simulink model "turbo_controller"  (R2025a)
settings: Solver=FixedStepAuto  StartTime=0.0  StopTime=inf  FixedStep=0.001  RelTol=1e-3
PostLoadFcn:
  | % 自动定位同目录CubeMX文件；不需要外部初始化脚本。
  | codertarget.data.setParameterValue('turbo_controller','STM32CubeMX.ProjectFile',fullfile(fileparts(get_param('turbo_controller','FileName')),'turbo_f407.ioc'));
InitFcn:
  | % 中文说明：按原控制器字段与类型创建三组接口总线；控制参数已内嵌。
  | tc_names=["EValve_Cycle" "EValve_Open" "Eblast_Cycle" "Eblast_Open" "Motor_Cycle" "Motor_Open" "EValve_Enable" "Eblast_Enable" "Motor_Enable" "SWO_Firework" "SWO_BleedAir" "EngineState" "Flag_ECUReset_Clear" "Flag_ECUReset_Save" "Flag_Reset_Enable" "Accelerator" "Nc_dem" "Nc"]; tc_types=["uint16" "uint16" "uint16" "uint16" "uint16" "uint16" "uint8" "uint8" "uint8" "uint8" "uint8" "uint8" "uint8" "uint8" "uint8" "single" "single" "single"];
  | for tc_k=1:numel(tc_names)
  |  tc_e(tc_k)=Simulink.BusElement; tc_e(tc_k).Name=char(tc_names(tc_k)); tc_e(tc_k).DataType=char(tc_types(tc_k));
  | end
  | EngineControl_Out=Simulink.Bus; EngineControl_Out.DataScope='Exported'; EngineControl_Out.Elements=tc_e;
  | clear tc_e tc_names tc_types tc_k
  | tc_names=["savedata1" "savedata2" "savedata3" "savedata4" "savedata5" "savedata6" "savedata7" "savedata8" "savedata9" "savedata10" "savedata11" "savedata12" "savedata13" "savedata14" "savedata15" "savedata16" "savedata17" "savedata18" "savedata19" "savedata20" "savedata21" "savedata22" "savedata23" "savedata24" "savedata25"]; tc_types=["single" "single" "single" "single" "single" "single" "single" "single" "single" "single" "single" "single" "single" "single" "single" "single" "single" "single" "single" "single" "single" "single" "single" "single" "single"];
  | for tc_k=1:numel(tc_names)
  |  tc_e(tc_k)=Simulink.BusElement; tc_e(tc_k).Name=char(tc_names(tc_k)); tc_e(tc_k).DataType=char(tc_types(tc_k));
  | end
  | SaveData_Out=Simulink.Bus; SaveData_Out.DataScope='Exported'; SaveData_Out.Elements=tc_e;
  | clear tc_e tc_names tc_types tc_k
  | tc_names=["senddata1" "senddata2" "senddata3" "senddata4" "senddata5" "senddata6" "senddata7" "senddata8" "senddata9" "senddata10" "senddata11" "senddata12" "senddata13" "senddata14" "senddata15" "senddata16" "senddata17" "senddata18" "senddata19" "senddata20" "senddata21" "senddata22" "senddata23" "senddata24" "senddata25" "senddata26" "senddata27" "senddata28" "senddata29"]; tc_types=["uint8" "uint8" "uint8" "uint8" "uint8" "uint8" "uint8" "uint8" "uint8" "uint8" "uint8" "uint8" "uint8" "uint8" "uint8" "uint8" "uint8" "uint8" "uint8" "uint8" "uint8" "uint8" "uint8" "uint8" "uint8" "uint8" "uint8" "uint8" "uint8"];
  | for tc_k=1:numel(tc_names)
  |  tc_e(tc_k)=Simulink.BusElement; tc_e(tc_k).Name=char(tc_names(tc_k)); tc_e(tc_k).DataType=char(tc_types(tc_k));
  | end
  | SendData_Out=Simulink.Bus; SendData_Out.DataScope='Exported'; SendData_Out.Elements=tc_e;
  | clear tc_e tc_names tc_types tc_k
  | 
  | % 以下为接口中文说明；只设置描述，不改变数值或数据类型。
  | EngineControl_Out.Description='执行控制输出（阀、电机、点火、状态及复位请求）';
  | tc_cn=["EValve_Cycle（主油阀周期计数（每计数2毫秒））" "EValve_Open（主油阀开通计数（每计数2毫秒））" "Eblast_Cycle（副油阀周期计数（每计数2毫秒））" "Eblast_Open（副油阀开通计数（每计数2毫秒））" "Motor_Cycle（起动电机周期计数）" "Motor_Open（起动电机开通计数）" "EValve_Enable（主油阀驱动使能）" "Eblast_Enable（副油阀驱动使能）" "Motor_Enable（起动电机使能）" "SWO_Firework（点火器使能（1开））" "SWO_BleedAir（引气阀使能（1开））" "EngineState（发动机状态）" "Flag_ECUReset_Clear（清除复位恢复状态请求）" "Flag_ECUReset_Save（保存复位恢复数据请求）" "Flag_Reset_Enable（处理器软件复位请求）" "Accelerator（油门／油泵给定控制量）" "Nc_dem（控制目标转速）" "Nc（发动机反馈转速（转每分））"];
  | tc_elements=EngineControl_Out.Elements;
  | for tc_k=1:numel(tc_cn)
  |  tc_elements(tc_k).Description=char(tc_cn(tc_k));
  | end
  | EngineControl_Out.Elements=tc_elements;
  | clear tc_cn tc_elements tc_k
  | SaveData_Out.Description='25项运行记录；字段含义按当前模型数据来源解释';
  | tc_cn=["savedata1（指令回显记录）" "savedata2（入口总温记录（℃））" "savedata3（电源电压记录）" "savedata4（排气温度记录（℃））" "savedata5（标定燃油压力记录）" "savedata6（副油阀占空比记录（％））" "savedata7（主油阀占空比记录（％））" "savedata8（温度修正转速记录）" "savedata9（开关输出及反馈位域）" "savedata10（物理转速记录）" "savedata11（油泵目标给定原始值）" "savedata12（起动电机占空比记录（％））" "savedata13（发动机状态码记录）" "savedata14（故障告警位域记录）" "savedata15（模型记录帧序号）" "savedata16（处理器温度记录（℃））" "savedata17（装订转速记录（沿用旧电源字段名））" "savedata18（导航高度记录）" "savedata19（飞行空速记录）" "savedata20（主阀旧记录位（恒零保留））" "savedata21（第21项保留记录（恒零））" "savedata22（保留记录项22）" "savedata23（保留记录项23）" "savedata24（保留记录项24）" "savedata25（保留记录项25）"];
  | tc_elements=SaveData_Out.Elements;
  | for tc_k=1:numel(tc_cn)
  |  tc_elements(tc_k).Description=char(tc_cn(tc_k));
  | end
  | SaveData_Out.Elements=tc_elements;
  | clear tc_cn tc_elements tc_k
  | SendData_Out.Description='29字段回传及外设命令接口；板端上位机帧只取第3至27字段';
  | tc_cn=["senddata1（回传发送允许标志（不直接上线路））" "senddata2（回传载荷长度25字节）" "senddata3（回传指令回显字节）" "senddata4（总温编码字节（℃＋80））" "senddata5（电源电压编码字节）" "senddata6（排温编码高字节）" "senddata7（排温编码低字节）" "senddata8（燃油压力编码高字节）" "senddata9（燃油压力编码低字节）" "senddata10（副油阀占空比字节（％））" "senddata11（主油阀占空比字节（％））" "senddata12（修正转速编码高字节）" "senddata13（修正转速编码低字节）" "senddata14（驱动及反馈状态位域）" "senddata15（物理转速编码高字节）" "senddata16（物理转速编码低字节）" "senddata17（油泵目标给定高字节（串口二使用））" "senddata18（油泵目标给定低字节（串口二使用））" "senddata19（起动电机占空比命令（串口一使用））" "senddata20（发动机状态码字节）" "senddata21（故障告警位域字节）" "senddata22（帧序号占位（板端另行填写））" "senddata23（处理器温度编码（℃＋50））" "senddata24（控制目标转速编码高字节）" "senddata25（控制目标转速编码低字节）" "senddata26（占位字节（板端改填实测泵速高字节））" "senddata27（占位字节（板端改填实测泵速低字节））" "senddata28（装订转速高字节（本板未发送））" "senddata29（装订转速低字节（本板未发送））"];
  | tc_elements=SendData_Out.Elements;
  | for tc_k=1:numel(tc_cn)
  |  tc_elements(tc_k).Description=char(tc_cn(tc_k));
  | end
  | SendData_Out.Elements=tc_elements;
  | clear tc_cn tc_elements tc_k
  | 
  | 
  | % FRAM模块化事务：接口类型和上电初始状态，随模型保存，无外部初始化文件。
  | clear FM_elements
  | FM_elements(1)=Simulink.BusElement;FM_elements(1).Name='phase';FM_elements(1).DataType='uint8';FM_elements(1).Dimensions=[1 1];FM_elements(1).Description='phase（当前事务阶段）';
  | FM_elements(2)=Simulink.BusElement;FM_elements(2).Name='a';FM_elements(2).DataType='uint8';FM_elements(2).Dimensions=[64 1];FM_elements(2).Description='a（启动时缓存的首区64字节）';
  | FM_elements(3)=Simulink.BusElement;FM_elements(3).Name='active';FM_elements(3).DataType='uint16';FM_elements(3).Dimensions=[1 1];FM_elements(3).Description='active（当前有效记录区地址）';
  | FM_elements(4)=Simulink.BusElement;FM_elements(4).Name='generation';FM_elements(4).DataType='uint32';FM_elements(4).Dimensions=[1 1];FM_elements(4).Description='generation（当前有效记录代号）';
  | FM_elements(5)=Simulink.BusElement;FM_elements(5).Name='record';FM_elements(5).DataType='uint8';FM_elements(5).Dimensions=[64 1];FM_elements(5).Description='record（本次冻结的待写记录）';
  | FM_elements(6)=Simulink.BusElement;FM_elements(6).Name='addr';FM_elements(6).DataType='uint16';FM_elements(6).Dimensions=[1 1];FM_elements(6).Description='addr（本次备用写入地址）';
  | FM_elements(7)=Simulink.BusElement;FM_elements(7).Name='lastSave';FM_elements(7).DataType='single';FM_elements(7).Dimensions=[1 1];FM_elements(7).Description='lastSave（上次开始保存的秒数）';
  | FM_elements(8)=Simulink.BusElement;FM_elements(8).Name='lastState';FM_elements(8).DataType='uint8';FM_elements(8).Dimensions=[1 1];FM_elements(8).Description='lastState（上次保存时的发动机状态）';
  | FM_elements(9)=Simulink.BusElement;FM_elements(9).Name='boot';FM_elements(9).DataType='boolean';FM_elements(9).Dimensions=[1 1];FM_elements(9).Description='boot（启动记录是否允许恢复）';
  | FM_elements(10)=Simulink.BusElement;FM_elements(10).Name='consumed';FM_elements(10).DataType='boolean';FM_elements(10).Dimensions=[1 1];FM_elements(10).Description='consumed（本次启动恢复通知是否已发送）';
  | FM_elements(11)=Simulink.BusElement;FM_elements(11).Name='payload';FM_elements(11).DataType='uint8';FM_elements(11).Dimensions=[20 1];FM_elements(11).Description='payload（当前20字节恢复内容）';
  | ... (+35 lines)
model workspace (MAT data in the model file):
  CRC16_Table_Reference = [0 4129 8258 12387 16516 20645 24774 28903 33032 37161 41290 45419 ... (256 elements, 256x1)]
  PE_Kaer = [0.15402 0.15402 0.12264 0.10076 0.09481 0.07601 0.07111 0.0569 0.05198 0.04926 0.05308 0.04325 ... (13 elements, 1x13)]
  PE_Nr = [21.2982 61.4260372 67.7475458 72.7394382 76.845934 80.6988798 83.8449282 86.6491912 88.9382406 89.178606 91.1938214 93.4068058 ... (13 elements, 1x13)]
  PE_Pump_Translate = 33.5999984741
  PE_RotaSpeed_Translate = 860
  PE_Taer = [0.4939154 0.4939154 0.40780982 0.34066978 0.31622756 0.30405716 0.34300244 0.26785022 0.37393554 0.23914836 0.44563948 0.31044662 ... (13 elements, 1x13)]
  PF_ACCFULLRANGE = 3360
  PF_Flag_ECUReset = 0
  PF_Flag_rx_suc = 1
  PF_Gear_Info = [40000; 45000; 50000; 55000; 57000; 59000; 60000; 61000; 61000; 61000; 61000; 61000]
  PF_K_TiaoJie = 1
  PF_Kpu = 10
  PF_MySet_Rxdata = [0 0 0 0 0 0 0 0 0 0 0 0 ... (50 elements, 50x1)]
  PF_MyUsart1_Rxdata = [0 0 0 0 0 0 0 0 0 0 0 0 ... (50 elements, 50x1)]
  PF_MyUsart2_Rxdata = [0 0 0 0 0 0 0 0 0 0 0 0 ... (50 elements, 50x1)]
  PF_Reset_Information = [0 0 0 0 0 0 0 0 0 0 0 0 ... (20 elements, 20x1)]
  PF_Sensor_X1_T4 = [0 4095]
  PF_Sensor_X2_T4 = [0 1.66666698456]
  PF_Sensor_X3_T4 = [0 504 999 1497 2010 2529 3051 3568 4076 4571 4959]
  PF_Sensor_X_P2 = [0.5 3]
  PF_Sensor_X_Poil = [0.5 3]
  PF_Sensor_X_T1t = [-50 300]
  PF_Sensor_X_Vpower = [0 3]
  PF_Sensor_X_Vpump = [0 3]
  PF_Sensor_Y1_T4 = [0 3]
  PF_Sensor_Y2_T4 = [0 5000]
  PF_Sensor_Y3_T4 = [0 100 200 300 400 500 600 700 800 900 980]
  PF_Sensor_Y_P2 = [0 1000]
  PF_Sensor_Y_Poil = [0 1000]
  PF_Sensor_Y_T1t = [-50 300]
  PF_Sensor_Y_Vpower = [0 33]
  PF_Sensor_Y_Vpump = [0 33]
  PG_CtrlMode_CloseLoop : mpt.Parameter (value not decoded)
  PG_CtrlMode_ManualAcc : mpt.Parameter (value not decoded)
  PG_CtrlMode_Origin : mpt.Parameter (value not decoded)
  PG_CtrlMode_Start : mpt.Parameter (value not decoded)
  PG_CtrlMode_Stop : mpt.Parameter (value not decoded)
  PG_ES_Clp : mpt.Parameter (value not decoded)
  PG_ES_EngStart : mpt.Parameter (value not decoded)
  PG_ES_Manual : mpt.Parameter (value not decoded)
  PG_ES_Origin : mpt.Parameter (value not decoded)
  PG_ES_Stop : mpt.Parameter (value not decoded)
  PG_Instr_BleedAirSet : mpt.Parameter (value not decoded)
  PG_Instr_CloseLoop : mpt.Parameter (value not decoded)
  PG_Instr_ECUReSet : mpt.Parameter (value not decoded)
  PG_Instr_EValveSet : mpt.Parameter (value not decoded)
  PG_Instr_EblastSet : mpt.Parameter (value not decoded)
  PG_Instr_Erase : mpt.Parameter (value not decoded)
  PG_Instr_FireWorkSet : mpt.Parameter (value not decoded)
  PG_Instr_ManualPlus : mpt.Parameter (value not decoded)
  PG_Instr_ManualrReduce : mpt.Parameter (value not decoded)
  PG_Instr_MotorSet : mpt.Parameter (value not decoded)
  PG_Instr_OilSet : mpt.Parameter (value not decoded)
  PG_Instr_SelfCheck : mpt.Parameter (value not decoded)
  PG_Instr_Start : mpt.Parameter (value not decoded)
  PG_Instr_Stop : mpt.Parameter (value not decoded)
  PG_Instr_StopZero : Simulink.Parameter (value not decoded)
  PG_Location_Air : Simulink.Parameter (value not decoded)
  PG_Location_Gnd : Simulink.Parameter (value not decoded)
  PG_ServoCtrlMode_CloseLoop : Simulink.Parameter (value not decoded)
  PG_ServoCtrlMode_CloseLoopMax : Simulink.Parameter (value not decoded)
  PG_ServoCtrlMode_CloseLoopMin : Simulink.Parameter (value not decoded)
  PG_ServoCtrlMode_ManualAcc : Simulink.Parameter (value not decoded)
  PG_ServoCtrlMode_ManualAccMax : Simulink.Parameter (value not decoded)
  PG_ServoCtrlMode_ManualAccMin : Simulink.Parameter (value not decoded)
  PG_SpeedDot_Permit : Simulink.Parameter (value not decoded)
  PL_EngineModel_Actuator = [0 10 100]
  PL_EngineModel_EngineStar_Press_P2 = [1013 1098.4 1099.144828 1099.931034 1103.613793 1162.662069 1143.793103 1131.006897 1123.186207 1117.6 1114 1111.806897 ... (127 elements, 1x127)]
  PL_EngineModel_EngineStar_RotaSpeed = [200 2000 9584 9660 10220 10240 10260 10288 10308 10368 10380 10408 ... (127 elements, 1x127)]
  PL_EngineModel_EngineStar_Temp_Exhaust = [128 129 129.1 130 131 131.1 132 133 134 134.1 135 135.1 ... (127 elements, 1x127)]
  PL_EngineModel_EngineStar_Time = [0.05 0.1 0.15 0.2 0.25 0.3 0.35 0.4 0.45 0.5 0.55 0.6 ... (127 elements, 1x127)]
  PL_EngineModel_IdleAbove_Nr = [0 21.2982 61.4260372 67.7475458 72.7394382 76.845934 80.6988798 83.8449282 86.6491912 88.9382406 89.178606 91.1938214 ... (14 elements, 1x14)]
  PL_EngineModel_IdleAbove_P2r = [0.986923266716 1.57907722675 1.81593881076 1.99358499877 2.23044658278 2.43770046879 2.65482358747 2.84233900814 3.03972366149 3.18776215149 3.25684678016 3.3950160375 ... (14 elements, 1x14)]
  PL_EngineModel_IdleAbove_Tempr = [0.0536001429337 1.07200285867 1.63301768805 1.63659103091 1.66875111667 1.72592460247 1.77595140254 1.86171163123 1.95461854565 2.03323208862 2.03323208862 2.13685903162 ... (14 elements, 1x14)]
  PL_EngineModel_IdleAbove_Ter = [0.42434128 0.42434128 0.42434128 0.30669408 0.23570008 0.22150128 0.1997974 0.23803274 0.16115638 0.24279948 0.13600422 0.31308354 ... (14 elements, 1x14)]
  PL_EngineModel_IdleAbove_Wfr = [0 10.142 23.8337 27.8905 31.9473 36.0041 40.0609 44.1177 48.1745 52.2313 52.7384 56.7952 ... (14 elements, 1x14)]
  PL_EngineModel_Press_P2 = [400 400 400 400 400 400 400 400 400 400]
  PL_EngineModel_Rotaspeed = [0 20000 96400]
  PL_EngineModel_Temp_Exhaust = [500 500 500 500 500 500 500 500 500 500]
  PL_Kaer = [0.1 0.1 0.1 0.1 0.1 0.1]
  PL_Nr = [50 60 70 80 90 100]
  PL_Taer = [0.1 0.1 0.1 0.1 0.1 0.1]
  Sig : Simulink.Signal (value not decoded)
  Ts_ms : Simulink.Parameter (value not decoded)
  false : Simulink.Parameter (value not decoded)
  true : Simulink.Parameter (value not decoded)
symbols that are objects in the model workspace (value not decoded): PG_CtrlMode_CloseLoop, PG_CtrlMode_ManualAcc, PG_CtrlMode_Origin, PG_CtrlMode_Start, PG_CtrlMode_Stop, PG_ES_Clp, PG_ES_EngStart, PG_ES_Manual, PG_ES_Origin, PG_ES_Stop, PG_Instr_BleedAirSet, PG_Instr_CloseLoop, PG_Instr_EblastSet, PG_Instr_ECUReSet, PG_Instr_Erase, PG_Instr_EValveSet, PG_Instr_FireWorkSet, PG_Instr_ManualPlus, PG_Instr_ManualrReduce, PG_Instr_MotorSet, PG_Instr_OilSet, PG_Instr_SelfCheck, PG_Instr_Start, PG_Instr_Stop, PG_Instr_StopZero, PG_ServoCtrlMode_CloseLoop, PG_ServoCtrlMode_CloseLoopMax, PG_ServoCtrlMode_CloseLoopMin, PG_ServoCtrlMode_ManualAcc, PG_ServoCtrlMode_ManualAccMax, PG_ServoCtrlMode_ManualAccMin, Ts_ms
libraries: simulink x97, stm32blockslib x10, stm32f4xxblockslib x8
(part 13 of 26)

== system turbo_controller/CLM/ClpControl/CtrlLaw ==
  note: 增量PI怎样把转速偏差变成油泵给定
      |
      | 输入包含当前目标、实际滤波转速、允许误差、Kp/Ki，以及上一周期油泵给定u_last。先求本次误差e
      | =目标-反馈，Time Delay8保存上次误差e_prev。
      |
      | 原始增量为：
      | Δu_raw=PF_K_TiaoJie×[Kp×(e-e_prev)+Ki×e]；
      | 当前PF_K_TiaoJie为1。Kp看误差变化，Ki看本次误差。这里已经是离散增量形式，不能再凭名称额外
      | 乘一次采样时间。
      |
      | 入口总压先限在30～100，再除100得到q。增量限制在-10q～+10q之间，压力低时允许步长也变小。
      | 若abs(e)小于允许值300，输出直接保持u_last；否则输出u_last+限幅后的Δu。另一路S_Step_Accler
      | ator输出这次限幅增量供记录/参数使用。
      |
      | 例如q=1、计算增量为25，实际只加10；误差已在300以内时，即使算出小增量也采用保持支路。
      | 结果随后仍经过Fault_Process和模式仲裁，不能把本层候选给定当作已发送到油泵的最终命令。
  S_Acclerator_Last : Inport
      settings: AttributesFormatString=S_Acclerator_Last（油门上一周期）
  S_RotaSpeed_ErrorAllow : Inport  Port=2
      settings: AttributesFormatString=S_RotaSpeed_ErrorAllow（转速误差或异常允许）
  S_Kp : Inport  Port=3
      settings: AttributesFormatString=S_Kp（比例系数）
  S_Ki : Inport  Port=4
      settings: AttributesFormatString=S_Ki（积分系数）
  S_Nc_dem : Inport  Port=5
      settings: AttributesFormatString=S_Nc_dem（控制目标转速）
  S_Nc_Filter : Inport  Port=6
      settings: AttributesFormatString=S_Nc_Filter（滤波后的转速）
  SPM : Inport  Port=7
      settings: AttributesFormatString=SPM（通信及传感器信息总线）
  Abs : Abs  SaturateOnIntegerOverflow=off
      settings: AttributesFormatString=Abs（绝对值）
  Bus Selector2 : BusSelector  OutputSignals=COMM（通信信息总线）.P1t_calc（入口总压计算值）
      settings: AttributesFormatString=Bus Selector2（总线选择器2）
  Constant7 : Constant  Value=PF_K_TiaoJie  OutDataTypeStr=single  SampleTime=-1
      settings: AttributesFormatString=Constant7（常量7）
  Product{1..3,5..7,11} (7 alike) : Product  Inputs=**
      Product1 settings: AttributesFormatString=Product1（乘法1）
      Product11 settings: AttributesFormatString=Product11（乘法11）
      Product2 settings: AttributesFormatString=Product2（乘法2）
      Product3 settings: AttributesFormatString=Product3（乘法3）
      Product5 settings: AttributesFormatString=Product5（乘法5）
      Product6 settings: AttributesFormatString=Product6（乘法6）
      Product7 settings: AttributesFormatString=Product7（乘法7）
  Product4 : Product  Inputs=*/
      settings: AttributesFormatString=Product4（乘法4）
  Range : Stateflow chart  Description=|  TreatAsAtomicUnit=on
      | 本实例限制PI每拍计算的泵给定增量，上下限为±10×q，其中q=限幅后的入口总压/100，q在0.3～1之间。例如q=0.5时只允许本拍增加或减少5。
      | 
      | 把一个数限制在允许范围内
      | 
      | 输入包括待处理值、允许下限和允许上限。先比较是否越过上限，越过就输出上限；未超过上限时再检查下限，小于下限就输出下限；落在范围内则原样通过。恰好等于边界的值也保留。
      | 
      | 计算式：输出 = min(max(输入，下限)，上限)。
      | 例如下限为0、上限为100时，输入120输出100，输入-5输出0，输入60输出60。这里不做平均、不计算变化速度，也不记住上一拍；它只防止当前数值越界。具体边界由父子系统连入，不能把此处的输出一律理解为百分比。
      settings: AttributesFormatString=Range（限幅或范围）
  Range1 : Stateflow chart  Description=|  TreatAsAtomicUnit=on
      | 本实例把通信入口总压P1t_calc限制在30～100，再除以100得到PI步长修正系数q。例如入口总压20先变30，q=0.3；入口总压80得到q=0.8。
      | 
      | 把一个数限制在允许范围内
      | 
      | 输入包括待处理值、允许下限和允许上限。先比较是否越过上限，越过就输出上限；未超过上限时再检查下限，小于下限就输出下限；落在范围内则原样通过。恰好等于边界的值也保留。
      | 
      | 计算式：输出 = min(max(输入，下限)，上限)。
      | 例如下限为0、上限为100时，输入120输出100，输入-5输出0，输入60输出60。这里不做平均、不计算变化速度，也不记住上一拍；它只防止当前数值越界。具体边界由父子系统连入，不能把此处的输出一律理解为百分比。
      settings: AttributesFormatString=Range1（限幅或范围1）
  Relational Operator : RelationalOperator  Operator=<  OutDataTypeStr=boolean  InputSameDT=off
      settings: AttributesFormatString=Relational Operator（关系比较运算）
  Sum of Elements : Sum
      settings: AttributesFormatString=Sum of Elements（加法求和的元素）
  Sum1 : Sum  Inputs=|+-
      settings: AttributesFormatString=Sum1（加法求和1）
  Sum2 : Sum  Inputs=|++
      settings: AttributesFormatString=Sum2（加法求和2）
  Sum3 : Sum  Inputs=|+-
      settings: AttributesFormatString=Sum3（加法求和3）
  Switch : Switch  Criteria=u2 ~= 0  SaturateOnIntegerOverflow=off  InputSameDT=off
      settings: AttributesFormatString=Switch（开关选择）
  Time Delay8 : UnitDelay  SampleTime=-1  HasFrameUpgradeWarning=on
      settings: AttributesFormatString=Time Delay8（时间延迟8）
  dth = T0-288.1 : Constant  OutDataTypeStr=single  SampleTime=-1
      settings: AttributesFormatString=dth = T0-288.1（固定常量1（旧名称不参与计算））
  dth = T0-288.2 : Constant  Value=100  OutDataTypeStr=single  SampleTime=-1
      settings: AttributesFormatString=dth = T0-288.2（固定常量100（旧名称不参与计算））
  dth = T0-288.3 : Constant  Value=100  OutDataTypeStr=single  SampleTime=-1
      settings: AttributesFormatString=dth = T0-288.3（固定常量100（旧名称不参与计算））
  dth = T0-288.4 : Constant  Value=10  OutDataTypeStr=single  SampleTime=-1
      settings: AttributesFormatString=dth = T0-288.4（固定常量10（旧名称不参与计算））
  dth = T0-288.5 : Constant  Value=30  OutDataTypeStr=single  SampleTime=-1
      settings: AttributesFormatString=dth = T0-288.5（固定常量30（旧名称不参与计算））
  dth = T0-288.6 : Constant  Value=-10  OutDataTypeStr=single  SampleTime=-1
      settings: AttributesFormatString=dth = T0-288.6（固定常量-10（旧名称不参与计算））
  S_CloseLoop_Acclerator : Outport
      settings: AttributesFormatString=S_CloseLoop_Acclerator（闭合回路油门）
  S_Step_Acclerator : Outport  Port=2
      settings: AttributesFormatString=S_Step_Acclerator（阶跃或步进油门）
  wires:
  S_RotaSpeed_ErrorAllow/1 -> Relational Operator/2
  S_Nc_Filter/1 -> [Nc_Filter]
  Range/1(Out) -> Sum2/2, S_Step_Acclerator/1
  [Nc_Filter] -> Sum1/2
  S_Nc_dem/1 -> [Nc_dem]
  Sum1/1 -> Time Delay8/1, Sum3/1, Abs/1, Product3/1
  [Nc_dem] -> Sum1/1
  dth = T0-288.2/1 -> Product4/2
  Product6/1 -> Product2/2
  Abs/1 -> Relational Operator/1
  Product11/1 -> Range/2(Max)
  Time Delay8/1 -> Sum3/2
  S_Kp/1 -> Product6/1
  Constant7/1 -> Product6/2, Product7/2
  S_Ki/1 -> Product7/1
  SPM/1 -> Bus Selector2/1
  Relational Operator/1 -> Switch/2
  Sum3/1 -> Product2/1
  dth = T0-288.4/1 -> Product11/1
  Product7/1 -> Product3/2
  Bus Selector2/1 -> Range1/1(In)  "<P1t_calc（入口总压计算值）>"
  dth = T0-288.3/1 -> Range1/2(Max)
  dth = T0-288.5/1 -> Range1/3(Min)
  Product2/1 -> Sum of Elements/1
  Product3/1 -> Sum of Elements/2
  Range1/1(Out) -> Product4/1
  Sum of Elements/1 -> Product1/1
  dth = T0-288.1/1 -> Product1/2
  Product4/1 -> Product11/2, Product5/2
  dth = T0-288.6/1 -> Product5/1
  Product1/1 -> Range/1(In)
  Product5/1 -> Range/3(Min)
  S_Acclerator_Last/1 -> Switch/1, Sum2/1
  Sum2/1 -> Switch/3
  Switch/1 -> S_CloseLoop_Acclerator/1

== system turbo_controller/CLM/ClpControl/Fault_Process ==
  note: 详细中文说明（1/1）
      | turbo_controller:533072
      | 【中文学习说明】D9-Nr-T5r
      | 一、它是做什么的？
      | 根据转速与高度做二维插值，计算故障处理需要的参数。先在各高度对应的一维转速曲
      | 线上插值，再按高度在两条结果间线性插值；原函数允许超出曲线范围时线性外推。输
      | 出是控制参数，不是新的传感器测量值。
      | 二、输入和输出怎么理解？
      | 输入接口：
      | 第1路 u1（输入一）。
      | 第2路 u2（输入二）。
      | 第3路 xin1（第一横坐标）。
      | 第4路 yin1（第一纵坐标）。
      | 第5路 xin2（第二横坐标）。
      | 第6路 yin2（第二纵坐标）。
      | 第7路 xin3（第三横坐标）。
      | 第8路 yin3（第三纵坐标）。
      | 输出接口：
      | 第1路 y（输出）。
      | 三、内部怎样一步步处理？
      | 四、时间、记忆与容易看错的地方
      | 学习顺序：先认本页任务与接口，再追踪条件和候选值，最后看输出来源。本文仅为说
      | 明，数值阈值、执行顺序和控制动作均由原图及参数决定。
  note: 转速故障时油泵给定怎样切换
      |
      | 本模块有正常PI候选值、上一周期油泵给定、转速故障Flag_NcFailure和锁存标志Lock_NcFailure，以
      | 及装订转速和高度。
      | 正常没有故障时，采用CtrlLaw的PI结果。
      |
      | Flag_NcFailure成立但尚未锁存时，先保持上次给定，避免可疑转速让PI继续乱调。Lock_NcFailure成
      | 立时，改用D9-Nr-T5r生成的备用给定，优先级高于前面的普通保持选择。
      |
      | 备用给定用装订转速和高度插值。三条高度曲线分别在40000与62000间给出对应给定：[2028,7342]、[
      | 1317,4148]、[702,1929]。高度先从m除1000转成km。结果再经GeneralFilter限到传入上下限，并按每
      | 次10的步长接近旧给定。
      |
      | 因此故障锁存后不是凭空把油泵清零，而是走预设的备用控制曲线。最终仍交ControlOut_Manage按控
      | 制模式与边界统一仲裁。
  note: D9-Nr-T5r
      | 按转速和高度插出备用油泵给定
      |
      | 父级传入装订转速N、以km表示的高度H，以及三条高度层曲线的转速断点和给定表。每条曲线先用inte
      | rp1按N线性插值，获得该高度层的给定；代码采用linear和extrap，超出转速断点时允许线性外推。
      |
      | 随后再按高度插值：H<5 km时，在0与5 km曲线结果之间插；H>=5 km时，在5与10 km曲线结果之间插。
      | 例如H=2.5 km，输出是0和5 km两条曲线给定的中点；H=7.5 km则取5和10 km结果的中点。
      |
      | 公式可写为：
      | 低层：u=u0+(u5-u0)×H/5；
      | 高层：u=u5+(u10-u5)×(H-5)/5。
      | 高度超出0～10 km时，公式仍会外推，并不自动按端点截住。
      |
      | 输出是转速故障备用给定，先交父级GeneralFilter限制幅值和每次变化量，再由故障标志决定是否采
      | 用。它不是新增的温度测量，也不替代真实转速采集。
  S_FAM : Inport
      settings: AttributesFormatString=S_FAM（故障标志总线）
  S_Acclerator_Last : Inport  Port=2
      settings: AttributesFormatString=S_Acclerator_Last（油门上一周期）
  S_CloseLoop_Acclerator : Inport  Port=3
      settings: AttributesFormatString=S_CloseLoop_Acclerator（闭合回路油门）
  SPM : Inport  Port=4
      settings: AttributesFormatString=SPM（通信及传感器信息总线）
  Acc_Min : Inport  Port=5
      settings: AttributesFormatString=Acc_Min（油门下限）
  Acc_Max : Inport  Port=6
      settings: AttributesFormatString=Acc_Max（油门上限）
  Bus Selector1 : BusSelector  OutputSignals=COMM（通信信息总线）.SpeedLoad（装订转速）,COMM（通信信息总线）.H_Gprs（导航高度）
      settings: AttributesFormatString=Bus Selector1（总线选择器1）
  Bus Selector3 : BusSelector  OutputSignals=Flag_NcFailure（转速传感器故障标志）,Lock_NcFailure（转速故障锁存）
      settings: AttributesFormatString=Bus Selector3（总线选择器3）
  D9-Nr-T5r : MATLAB Function  Description=|  TreatAsAtomicUnit=on
      | 按转速和高度插出备用油泵给定
      | 
      | 父级传入装订转速N、以km表示的高度H，以及三条高度层曲线的转速断点和给定表。每条曲线先用interp1按N线性插值，获得该高度层的给定；代码采用linear和extrap，超出转速断点时允许线性外推。
      | 
      | 随后再按高度插值：H<5 km时，在0与5 km曲线结果之间插；H>=5 km时，在5与10 km曲线结果之间插。
      | 例如H=2.5 km，输出是0和5 km两条曲线给定的中点；H=7.5 km则取5和10 km结果的中点。
      | 
      | 公式可写为：
      | 低层：u=u0+(u5-u0)×H/5；
      | 高层：u=u5+(u10-u5)×(H-5)/5。
      | 高度超出0～10 km时，公式仍会外推，并不自动按端点截住。
      | 
      | 输出是转速故障备用给定，先交父级GeneralFilter限制幅值和每次变化量，再由故障标志决定是否采用。它不是新增的温度测量，也不替代真实转速采集。
      settings: AttributesFormatString=D9-Nr-T5r（转速与高度特性二维插值（沿用原模板名））
  Data Type Conversion : DataTypeConversion  OutDataTypeStr=single  SaturateOnIntegerOverflow=off  RndMeth=Floor
      settings: AttributesFormatString=Data Type Conversion（数据类型转换）
  Data Type Conversion1 : DataTypeConversion  OutDataTypeStr=single  SaturateOnIntegerOverflow=off  RndMeth=Floor
      settings: AttributesFormatString=Data Type Conversion1（数据类型转换1）
  GeneralFilter : Subsystem  Description=|  RequirementInfo={} %GIDa_15b32305_6be5_41da_881d_1e414d4491bf
      | 让故障备用给定不要一步跳太远
      | 
      | 输入Xin是备用插值给定，上下限由父级传入；Acclerator_Last是上一周期给定，Xdot_lim当前为每次10。这里的目标是平滑切到备用控制，不是测量信号滤波。
      | 
      | 先把Xin限制在给定上下限，得到目标。计算目标与旧给定的差，若差的绝对值小于20，直接保持旧值，避免微小来回调整。
      | 差值达到20及以上时，根据方向从旧值加或减Xdot_lim，也就是本工程每次移动10。
      | 
      | 例如旧给定1000、目标1100，本次先给1010；旧给定1000、目标1015，差值15小于20，则继续保持1000。这个模块没有按误差大小比例变化，也不是指数低通。
      | 
      | 父级只有Lock_NcFailure成立才采用这一路结果。它内部的Range负责幅值约束，本层的加减负责步长，两者不能混作一种限幅。
      settings: AttributesFormatString=GeneralFilter（通用滤波）
  N1r_idle1 : Constant  Value=[2028 7342]  OutDataTypeStr=single  SampleTime=-1
      settings: AttributesFormatString=N1r_idle1（一级转速归一化值慢车1）
  N1r_idle17 : Constant  Value=[40000 62000]  OutDataTypeStr=single  SampleTime=-1
      settings: AttributesFormatString=N1r_idle17（一级转速归一化值慢车17）
  N1r_idle2 : Constant  Value=[40000 62000]  OutDataTypeStr=single  SampleTime=-1
      settings: AttributesFormatString=N1r_idle2（一级转速归一化值慢车2）
  N1r_idle3 : Constant  Value=[1317 4148]  OutDataTypeStr=single  SampleTime=-1
      settings: AttributesFormatString=N1r_idle3（一级转速归一化值慢车3）
  N1r_idle4 : Constant  Value=[40000 62000]  OutDataTypeStr=single  SampleTime=-1
      settings: AttributesFormatString=N1r_idle4（一级转速归一化值慢车4）
  N1r_idle5 : Constant  Value=[702 1929]  OutDataTypeStr=single  SampleTime=-1
      settings: AttributesFormatString=N1r_idle5（一级转速归一化值慢车5）
  Product5 : Product  Inputs=*/
      settings: AttributesFormatString=Product5（乘法5）
  Switch : Switch  Criteria=u2 ~= 0  SaturateOnIntegerOverflow=off  InputSameDT=off
      settings: AttributesFormatString=Switch（开关选择）
  Switch1 : Switch  Criteria=u2 ~= 0  SaturateOnIntegerOverflow=off  InputSameDT=off
      settings: AttributesFormatString=Switch（开关选择）
  constant4 : Constant  Value=1000  OutDataTypeStr=double  SampleTime=-1
      settings: AttributesFormatString=constant4（常量4）
  dth = T0-288.9 : Constant  Value=10  OutDataTypeStr=single  SampleTime=-1
      settings: AttributesFormatString=dth = T0-288.9（固定常量10（旧名称不参与计算））
  S_CloseLoop_Acclera tor_Out : Outport
      settings: AttributesFormatString=S_CloseLoop_Acclera tor_Out（闭合回路油门原油门变量的拼写分段输出）
  wires:
  Bus Selector3/1 -> Switch/2  "<Flag_NcFailure（转速传感器故障标志）>"
  Switch1/1 -> S_CloseLoop_Acclera tor_Out/1
  SPM/1 -> Bus Selector1/1
  Bus Selector1/1 -> Data Type Conversion/1  "<SpeedLoad（装订转速）>"
  Product5/1 -> Data Type Conversion1/1
  constant4/1 -> Product5/2
  N1r_idle5/1 -> D9-Nr-T5r/8(yin3)
  N1r_idle4/1 -> D9-Nr-T5r/7(xin3)
  N1r_idle3/1 -> D9-Nr-T5r/6(yin2)
  N1r_idle2/1 -> D9-Nr-T5r/5(xin2)
  N1r_idle1/1 -> D9-Nr-T5r/4(yin1)
  N1r_idle17/1 -> D9-Nr-T5r/3(xin1)
  Bus Selector1/2 -> Product5/1  "<H_Gprs（导航高度）>"
  Data Type Conversion/1 -> D9-Nr-T5r/1(u1)
  Data Type Conversion1/1 -> D9-Nr-T5r/2(u2)
  D9-Nr-T5r/1(y) -> GeneralFilter/1(Xin)
  Acc_Max/1 -> GeneralFilter/2(X_ulim)
  Acc_Min/1 -> GeneralFilter/3(X_llim)
  dth = T0-288.9/1 -> GeneralFilter/4(Xdot_lim)
  S_FAM/1 -> Bus Selector3/1
  Bus Selector3/2 -> Switch1/2  "<Lock_NcFailure（转速故障锁存）>"
  S_CloseLoop_Acclerator/1 -> Switch/3
  S_Acclerator_Last/1 -> Switch/1, GeneralFilter/5(Acclerator_Last)
  GeneralFilter/1(S_Xout) -> Switch1/1
  Switch/1 -> Switch1/3

== system turbo_controller/CLM/ControlOut_Manage/Accelerator_Manage ==
  note: 油泵给定最终从哪一路选择
      |
      | 输入同时带有当前控制模式及五种模式的候选油泵值。ServoCtrlOut先按模式选择：原位取Vin_Origin
      | ，起动取Vin_Start，停车取Vin_Stop；闭环与手动则在各自最小/最大给定内限制候选值。
      |
      | 例如闭环候选9000而上限8000，输出8000，并把ServoCtrlFlag置为闭环上限分支；正常处于范围内时
      | 保留候选值。这个标志用于告诉后面“为什么给了这个值”。
      |
      | 图外LogicSelection3再看Flag_ECUReset_work：有效时采用恢复记录中的ECUReset_Acclerator，否则
      | 采用ServoCtrlOut的Vout。两层选择顺序不同，恢复支路是在模式选择之后。
      |
      | 输出一路是给定值，另一路是选择标志，随后组成执行总线。当前上层恢复许可接false，不能因这里
      | 保留了恢复选择接口就认定实机一定使用了恢复数据。
  S_FAM : Inport
      settings: AttributesFormatString=S_FAM（故障标志总线）
  S_CtrlMode : Inport  Port=2
      settings: AttributesFormatString=S_CtrlMode（控制模式）
  S_Origin_Accelerator : Inport  Port=3
      settings: AttributesFormatString=S_Origin_Accelerator（原位油门）
  S_Start_Accelerator : Inport  Port=4
      settings: AttributesFormatString=S_Start_Accelerator（起动油门）
  S_CloseLoop_Accelerator : Inport  Port=5
      settings: AttributesFormatString=S_CloseLoop_Accelerator（闭合回路油门）
  S_CloseLoop_CloseLoopMin : Inport  Port=6
      settings: AttributesFormatString=S_CloseLoop_CloseLoopMin（闭合回路闭合回路下限）
  S_CloseLoop_CloseLoopMax : Inport  Port=7
      settings: AttributesFormatString=S_CloseLoop_CloseLoopMax（闭合回路闭合回路上限）
  S_Stop_Accelerator : Inport  Port=8
      settings: AttributesFormatString=S_Stop_Accelerator（停车油门）
  S_Manual_Accelerator : Inport  Port=9
      settings: AttributesFormatString=S_Manual_Accelerator（手动油门）
  S_ManualAccMin : Inport  Port=10
      settings: AttributesFormatString=S_ManualAccMin（手动油门下限）
  S_ManualAccMax : Inport  Port=11
      settings: AttributesFormatString=S_ManualAccMax（手动油门上限）
  S_SPM : Inport  Port=12
      settings: AttributesFormatString=S_SPM（通信及传感器信息总线）
  Bus Selector1 : BusSelector  OutputSignals=Flag_ECUReset_work（复位恢复运行标志）
      settings: AttributesFormatString=Bus Selector1（总线选择器1）
  Bus Selector2 : BusSelector  OutputSignals=COMM（通信信息总线）.ECUReset_Acclerator（复位恢复油泵给定）
      settings: AttributesFormatString=Bus Selector2（总线选择器2）
  LogicSelection3 : Subsystem  Description=|
      | 复位恢复值是否覆盖普通油泵选择
      | 
      | 输入T是恢复记录的油泵给定，F是ServoCtrlOut按当前模式选出的普通给定，条件C来自Flag_ECUReset_work。
      | C非零时输出T；C为零时输出F。这里是一选一，不把两个给定相加，也不做渐变。
      | 
      | 例如普通给定1200、恢复值1500，许可成立时输出1500，否则1200。是否允许恢复由FPM和上游恢复解码链路决定；当前恢复许可有固定false的上游连接，不能仅凭本模块存在就认定恢复已启用。
      | 
      | 输出送本层统一油泵给定端口，然后再打包为执行总线。
      settings: AttributesFormatString=LogicSelection3（逻辑选择3）
  ServoCtrlOut : Stateflow chart  Description=|  TreatAsAtomicUnit=on
      | 按当前控制模式选择并限制油泵给定
      | 
      | EngineCtrlMode决定本次采用哪一种候选，不是比较几种候选谁最大。起动选Vin_Start，停车选Vin_Stop；不属于这些指定分支时走原位候选。
      | 
      | 闭环模式选Vin_Idle，但先限制在CloseLoopMin～CloseLoopMax；手动模式选Vin_Manual，限制在ManualAccMin～ManualAccMax。
      | 通用限幅关系为输出=min(max(候选,下限),上限)。
      | 
      | 每次选择还给出ServoCtrlFlag：例如闭环候选大于上限，就输出上限并标“闭环上限”；在范围内则标正常闭环。这样记录的不只是一个给定值，也能看出是否被限幅。
      | 
      | 本图没有低通滤波，也不直接发送串口命令。输出回到Accelerator_Manage后，外层还可能按复位恢复工作标志选择恢复给定。
      settings: AttributesFormatString=ServoCtrlOut（油泵给定选择）
  S_ServoCtrlFlag : Outport
      settings: AttributesFormatString=S_ServoCtrlFlag（油泵给定选择标志）
  S_Acclerator : Outport  Port=2
      settings: AttributesFormatString=S_Acclerator（油门／油泵给定控制量）
  wires:
  S_Origin_Accelerator/1 -> ServoCtrlOut/2(Vin_Origin)
  ServoCtrlOut/1(ServoCtrlFlag) -> S_ServoCtrlFlag/1
  LogicSelection3/1(Out) -> S_Acclerator/1
  ServoCtrlOut/2(Vout) -> LogicSelection3/3(F)
  S_FAM/1 -> Bus Selector1/1
  S_Start_Accelerator/1 -> ServoCtrlOut/3(Vin_Start)
  S_CloseLoop_Accelerator/1 -> ServoCtrlOut/4(Vin_Idle)
  S_CloseLoop_CloseLoopMin/1 -> ServoCtrlOut/5(CloseLoopMin)
  S_CloseLoop_CloseLoopMax/1 -> ServoCtrlOut/6(CloseLoopMax)
  S_Stop_Accelerator/1 -> ServoCtrlOut/7(Vin_Stop)
  S_Manual_Accelerator/1 -> ServoCtrlOut/8(Vin_Manual)
  S_ManualAccMin/1 -> ServoCtrlOut/9(ManualAccMin)
  S_ManualAccMax/1 -> ServoCtrlOut/10(ManualAccMax)
  S_CtrlMode/1 -> ServoCtrlOut/1(EngineCtrlMode)
  Bus Selector1/1 -> LogicSelection3/1(C)  "<Flag_ECUReset_work（复位恢复运行标志）>"
  S_SPM/1 -> Bus Selector2/1
  Bus Selector2/1 -> LogicSelection3/2(T)  "<ECUReset_Acclerator（复位恢复油泵给定）>"

== system turbo_controller/CLM/ControlOut_Manage/SWO_Manage ==
  note: 阀门电机等字段怎样随模式一起切换
      |
      | 油泵给定已经在同级Accelerator_Manage单独处理；本层负责其余执行机构字段。输入有原位、起动、
      | 闭环、手动、停车各模式总线，以及当前控制模式。
      |
      | Switch Case按模式只允许对应动作子系统运行，动作分支把那套周期、开启计数、使能、点火/引气等
      | 字段取出。Merge接收当前被执行分支的结果，不是把五个分支数值求和。
      |
      | 这样可以保证例如切入停车时，阀门和电机字段来自停车候选，而不是仍取起动分支保存的旧值。非当
      | 前分支可能保留历史输出，不能将保持值当作当前有效要求。
      |
      | 输出分别接入统一执行总线，再交ControlOut和BoardOutput。这里切换的是软件要求，2 ms阀门周期
      | 和1 ms点火节奏由板级输出层实现。
  S_CtrlMode : Inport
      settings: AttributesFormatString=S_CtrlMode（控制模式）
  S_Start : Inport  Port=2
      settings: AttributesFormatString=S_Start（地面起动）
  S_Origin : Inport  Port=3
      settings: AttributesFormatString=S_Origin（原位）
  S_Stop : Inport  Port=4
      settings: AttributesFormatString=S_Stop（停车）
  S_Manual : Inport  Port=5
      settings: AttributesFormatString=S_Manual（手动）
  S_CloseLoop : Inport  Port=6
      settings: AttributesFormatString=S_CloseLoop（闭合回路）
  Demux : Demux  Outputs=6
      settings: AttributesFormatString=Demux（信号分解）
  Demux1 : Demux  Outputs=5
      settings: AttributesFormatString=Demux1（信号分解1）
  Merge : Merge  Inputs=5
      settings: AttributesFormatString=Merge（条件分支输出合并）
  Merge1 : Merge  Inputs=5
      settings: AttributesFormatString=Merge1（条件分支输出合并1）
  Switch Case : SwitchCase  CaseConditions={PG_CtrlMode_Start,PG_CtrlMode_Stop,PG_CtrlMode_Origin,PG_CtrlMode_ManualAcc}
      settings: AttributesFormatString=Switch Case（开关选择分支情况）
  Switch Case Action Subsystem : Subsystem  Description=|  TreatAsAtomicUnit=on
      | 取出初始模式的阀门和电机控制量
      | 
      | 上层已根据发动机运行模式选中本分支。本分支不再判断是否允许起动或停车，而是把这一模式给出的11个控制字段分成两组，交给后面的输出管理。
      | 
      | 第一组是主油阀、副油阀和起动电机各自的“周期计数、开通计数”，共6项；第二组是这三个执行器的使能，以及点火器、引气阀的开关，共5项。这里的增益都为1，数值原样传递。
      | 
      | 周期计数不是毫秒。例如阀门周期30、开通15，只表示每30个输出节拍开15拍；到板级输出以2 ms节拍执行时才对应60 ms周期、30 ms开通。使能为0时，开通计数有值也不会实际驱动。输出分别汇入控制数值总线和使能总线。
      settings: AttributesFormatString=Switch Case Action Subsystem（开关分支动作子系统）
  Switch Case Action Subsystem1 : Subsystem  Description=|  TreatAsAtomicUnit=on
      | 取出起动模式的阀门和电机控制量
      | 
      | 上层已根据发动机运行模式选中本分支。本分支不再判断是否允许起动或停车，而是把这一模式给出的11个控制字段分成两组，交给后面的输出管理。
      | 
      | 第一组是主油阀、副油阀和起动电机各自的“周期计数、开通计数”，共6项；第二组是这三个执行器的使能，以及点火器、引气阀的开关，共5项。这里的增益都为1，数值原样传递。
      | 
      | 周期计数不是毫秒。例如阀门周期30、开通15，只表示每30个输出节拍开15拍；到板级输出以2 ms节拍执行时才对应60 ms周期、30 ms开通。使能为0时，开通计数有值也不会实际驱动。输出分别汇入控制数值总线和使能总线。
      settings: AttributesFormatString=Switch Case Action Subsystem1（开关分支动作子系统1）
  Switch Case Action Subsystem2 : Subsystem  Description=|  TreatAsAtomicUnit=on
      | 取出闭环模式的阀门和电机控制量
      | 
      | 上层已根据发动机运行模式选中本分支。本分支不再判断是否允许起动或停车，而是把这一模式给出的11个控制字段分成两组，交给后面的输出管理。
      | 
      | 第一组是主油阀、副油阀和起动电机各自的“周期计数、开通计数”，共6项；第二组是这三个执行器的使能，以及点火器、引气阀的开关，共5项。这里的增益都为1，数值原样传递。
      | 
      | 周期计数不是毫秒。例如阀门周期30、开通15，只表示每30个输出节拍开15拍；到板级输出以2 ms节拍执行时才对应60 ms周期、30 ms开通。使能为0时，开通计数有值也不会实际驱动。输出分别汇入控制数值总线和使能总线。
      settings: AttributesFormatString=Switch Case Action Subsystem2（开关分支动作子系统2）
  Switch Case Action Subsystem3 : Subsystem  Description=|  TreatAsAtomicUnit=on
      | 取出手动模式的阀门和电机控制量
      | 
      | 上层已根据发动机运行模式选中本分支。本分支不再判断是否允许起动或停车，而是把这一模式给出的11个控制字段分成两组，交给后面的输出管理。
      | 
      | 第一组是主油阀、副油阀和起动电机各自的“周期计数、开通计数”，共6项；第二组是这三个执行器的使能，以及点火器、引气阀的开关，共5项。这里的增益都为1，数值原样传递。
      | 
      | 周期计数不是毫秒。例如阀门周期30、开通15，只表示每30个输出节拍开15拍；到板级输出以2 ms节拍执行时才对应60 ms周期、30 ms开通。使能为0时，开通计数有值也不会实际驱动。输出分别汇入控制数值总线和使能总线。
      settings: AttributesFormatString=Switch Case Action Subsystem3（开关分支动作子系统3）
  Switch Case Action Subsystem4 : Subsystem  Description=|  TreatAsAtomicUnit=on
      | 取出停车模式的阀门和电机控制量
      | 
      | 上层已根据发动机运行模式选中本分支。本分支不再判断是否允许起动或停车，而是把这一模式给出的11个控制字段分成两组，交给后面的输出管理。
      | 
      | 第一组是主油阀、副油阀和起动电机各自的“周期计数、开通计数”，共6项；第二组是这三个执行器的使能，以及点火器、引气阀的开关，共5项。这里的增益都为1，数值原样传递。
      | 
      | 周期计数不是毫秒。例如阀门周期30、开通15，只表示每30个输出节拍开15拍；到板级输出以2 ms节拍执行时才对应60 ms周期、30 ms开通。使能为0时，开通计数有值也不会实际驱动。输出分别汇入控制数值总线和使能总线。
      settings: AttributesFormatString=Switch Case Action Subsystem4（开关分支动作子系统4）
  S_EValve_Cycle : Outport
      settings: AttributesFormatString=S_EValve_Cycle（主油阀周期计数（每计数2毫秒））
  S_EValve_Open : Outport  Port=2
      settings: AttributesFormatString=S_EValve_Open（主油阀开通计数（每计数2毫秒））
  S_Eblast_Cycle : Outport  Port=3
      settings: AttributesFormatString=S_Eblast_Cycle（副油阀周期计数（每计数2毫秒））
  S_Eblast_Open : Outport  Port=4
      settings: AttributesFormatString=S_Eblast_Open（副油阀开通计数（每计数2毫秒））
  S_Motor_Cycle : Outport  Port=5
      settings: AttributesFormatString=S_Motor_Cycle（起动电机周期计数）
  S_Motor_Open : Outport  Port=6
      settings: AttributesFormatString=S_Motor_Open（起动电机开通计数）
  S_EValve_Enable : Outport  Port=7
      settings: AttributesFormatString=S_EValve_Enable（主油阀驱动使能）
  S_Eblast_Enable : Outport  Port=8
      settings: AttributesFormatString=S_Eblast_Enable（副油阀驱动使能）
  S_Motor_Enable : Outport  Port=9
      settings: AttributesFormatString=S_Motor_Enable（起动电机使能）
  S_SWO_Firework : Outport  Port=10
      settings: AttributesFormatString=S_SWO_Firework（点火器使能（1开））
  S_SWO_BleedAir : Outport  Port=11
      settings: AttributesFormatString=S_SWO_BleedAir（引气阀使能（1开））
  wires:
  S_CtrlMode/1 -> Switch Case/1
  Switch Case Action Subsystem2/2(Out2) -> Merge1/2
  Switch Case Action Subsystem2/1(Out1) -> Merge/2
  S_Start/1 -> Switch Case Action Subsystem/1(In1)
  S_Manual/1 -> Switch Case Action Subsystem4/1(In1)
  S_Stop/1 -> Switch Case Action Subsystem2/1(In1)
  Switch Case/1 -> Switch Case Action Subsystem/Action
  Switch Case/2 -> Switch Case Action Subsystem2/Action
  Switch Case/3 -> Switch Case Action Subsystem1/Action
  Switch Case/4 -> Switch Case Action Subsystem4/Action
  Switch Case/5 -> Switch Case Action Subsystem3/Action
  S_Origin/1 -> Switch Case Action Subsystem1/1(In1)
  Demux/1 -> S_EValve_Cycle/1
  S_CloseLoop/1 -> Switch Case Action Subsystem3/1(In1)
  Switch Case Action Subsystem/2(Out2) -> Merge1/1
  Switch Case Action Subsystem/1(Out1) -> Merge/1
  Switch Case Action Subsystem1/2(Out2) -> Merge1/3
  Switch Case Action Subsystem1/1(Out1) -> Merge/3
  Switch Case Action Subsystem4/1(Out1) -> Merge/4
  Switch Case Action Subsystem4/2(Out2) -> Merge1/4
  Switch Case Action Subsystem3/2(Out3) -> Merge1/5
  Switch Case Action Subsystem3/1(Out2) -> Merge/5
  Merge/1 -> Demux/1
  Merge1/1 -> Demux1/1
  Demux/5 -> S_Motor_Cycle/1
  Demux/4 -> S_Eblast_Open/1
  Demux/3 -> S_Eblast_Cycle/1
  Demux/2 -> S_EValve_Open/1
  Demux1/1 -> S_EValve_Enable/1
  Demux/6 -> S_Motor_Open/1
  Demux1/5 -> S_SWO_BleedAir/1
  Demux1/4 -> S_SWO_Firework/1
  Demux1/3 -> S_Motor_Enable/1
  Demux1/2 -> S_Eblast_Enable/1

== system turbo_controller/CLM/Manual/BleedAir_Control ==
  note: 手动设置引气阀，其他命令不改它
      |
      | 同时满足“收到有效帧”和“命令为引气阀设置”时，读取Data6：Data6≥1输出开，Data6<1输出关。
      | 这里采用开关含义，不把Data6当成开度百分比。
      |
      | 条件不满足时，从上一拍控制输出总线取回SWO_BleedAir，保持原来的引气阀状态。因此发送油泵命令
      | 不会顺带关闭引气阀。该结果随后进入统一开关量输出，由板级输出转换成硬件电平。
  S_Flag_rs_suc : Inport
      settings: AttributesFormatString=S_Flag_rs_suc（标志接收状态成功或有效）
  S_Instr : Inport  Port=2
      settings: AttributesFormatString=S_Instr（指令）
  S_COMM_Data6 : Inport  Port=3
      settings: AttributesFormatString=S_COMM_Data6（通信数据6）
  S_ServoOut_Last : Inport  Port=4
      settings: AttributesFormatString=S_ServoOut_Last（伺服输出上一周期）
  Bus Selector2 : BusSelector  OutputSignals=SWO_BleedAir（引气阀使能）
      settings: AttributesFormatString=Bus Selector2（总线选择器2）
  Constant8 : Constant  OutDataTypeStr=uint8
      settings: AttributesFormatString=Constant8（常量8）
  Data Type Conversion1 : DataTypeConversion  OutDataTypeStr=uint8  SaturateOnIntegerOverflow=off  RndMeth=Floor
      settings: AttributesFormatString=Data Type Conversion1（数据类型转换1）
  Logical Operator : Logic  AllPortsSameDT=off  OutDataTypeStr=boolean
      settings: AttributesFormatString=Logical Operator（逻辑运算）
  N1r_idle1 : Constant  Value=PG_Instr_BleedAirSet  OutDataTypeStr=single  SampleTime=-1
      settings: AttributesFormatString=N1r_idle1（一级转速归一化值慢车1）
  Relational Operator1 : RelationalOperator  Operator===  OutDataTypeStr=boolean  InputSameDT=off
      settings: AttributesFormatString=Relational Operator1（关系比较运算1）
  Relational Operator2 : RelationalOperator  OutDataTypeStr=boolean  InputSameDT=off
      settings: AttributesFormatString=Relational Operator2（关系比较运算2）
  Switch : Switch  Criteria=u2 ~= 0  SaturateOnIntegerOverflow=off  InputSameDT=off
      settings: AttributesFormatString=Switch（开关选择）
  S_SWO_BleedAirSet : Outport
      settings: AttributesFormatString=S_SWO_BleedAirSet（输出引气空中或空气设置）
  wires:
  S_Instr/1 -> Relational Operator1/2
  S_Flag_rs_suc/1 -> Logical Operator/2
  N1r_idle1/1 -> Relational Operator1/1
  Relational Operator1/1 -> Logical Operator/1
  Switch/1 -> S_SWO_BleedAirSet/1
  Relational Operator2/1 -> Data Type Conversion1/1
  S_COMM_Data6/1 -> Relational Operator2/1
  Bus Selector2/1 -> Switch/3  "<SWO_BleedAir（引气阀使能）>"
  Constant8/1 -> Relational Operator2/2
  S_ServoOut_Last/1 -> Bus Selector2/1
  Data Type Conversion1/1 -> Switch/1
  Logical Operator/1 -> Switch/2

== system turbo_controller/CLM/Manual/Eblast_Control ==
  note: 把手动油阀开度换算为周期内的开通拍数
      |
      | 先确认有效帧属于本阀的设置命令，再把命令数据Data6按百分数换算：开通计数 = Data6×30/100，并
      | 限制在0～30；周期固定为30。例：Data6=50得到开通15拍，Data6=100得到开通30拍。
      |
      | 使能判断使用换算后的计数是否大于等于1，因此非常小的设定可能仍不使能阀门。没有本阀的新有效
      | 设置时，保持原设定。本处只生成周期、开通和使能三项，实际的2 ms输出节拍在板级输出中执行。
      |
      | 若阀门周期30、开通15，在2 ms节拍下就是每60 ms开30 ms。不要把这里的“15”直接读成15 ms。
  S_Flag_rs_suc : Inport
      settings: AttributesFormatString=S_Flag_rs_suc（标志接收状态成功或有效）
  S_Instr : Inport  Port=2
      settings: AttributesFormatString=S_Instr（指令）
  S_COMM_Data6 : Inport  Port=3
      settings: AttributesFormatString=S_COMM_Data6（通信数据6）
  Constant1 : Constant  Value=0  OutDataTypeStr=single
      settings: AttributesFormatString=Constant1（常量1）
  Constant2 : Constant  Value=100  OutDataTypeStr=single
      settings: AttributesFormatString=Constant2（常量2）
  Constant3 : Constant  Value=30  OutDataTypeStr=single
      settings: AttributesFormatString=Constant3（常量3）
  Constant5 : Constant  Value=30  OutDataTypeStr=uint16
      settings: AttributesFormatString=Constant5（常量5）
  Constant7 : Constant  Value=30  OutDataTypeStr=single
      settings: AttributesFormatString=Constant7（常量7）
  Constant8 : Constant  OutDataTypeStr=single
      settings: AttributesFormatString=Constant8（常量8）
  Data Type Conversion1 : DataTypeConversion  OutDataTypeStr=uint16  SaturateOnIntegerOverflow=off  RndMeth=Floor
      settings: AttributesFormatString=Data Type Conversion1（数据类型转换1）
  Data Type Conversion2 : DataTypeConversion  OutDataTypeStr=single  SaturateOnIntegerOverflow=off  RndMeth=Floor
      settings: AttributesFormatString=Data Type Conversion2（数据类型转换2）
  Data Type Conversion3 : DataTypeConversion  OutDataTypeStr=uint8  SaturateOnIntegerOverflow=off  RndMeth=Floor
      settings: AttributesFormatString=Data Type Conversion3（数据类型转换3）
  Logical Operator : Logic  AllPortsSameDT=off  OutDataTypeStr=boolean
      settings: AttributesFormatString=Logical Operator（逻辑运算）
  N1r_idle1 : Constant  Value=PG_Instr_EblastSet  OutDataTypeStr=single  SampleTime=-1
      settings: AttributesFormatString=N1r_idle1（一级转速归一化值慢车1）
  Product3 : Product  Inputs=*/*
      settings: AttributesFormatString=Product3（乘法3）
  Range : Stateflow chart  Description=|  TreatAsAtomicUnit=on
      | 本实例限制副油阀开通计数0～30，对应固定周期30。计算值45限制为30，最多整个周期都开，不会出现开通时间大于周期。
      | 
      | 把一个数限制在允许范围内
      | 
      | 输入包括待处理值、允许下限和允许上限。先比较是否越过上限，越过就输出上限；未超过上限时再检查下限，小于下限就输出下限；落在范围内则原样通过。恰好等于边界的值也保留。
      | 
      | 计算式：输出 = min(max(输入，下限)，上限)。
      | 例如下限为0、上限为100时，输入120输出100，输入-5输出0，输入60输出60。这里不做平均、不计算变化速度，也不记住上一拍；它只防止当前数值越界。具体边界由父子系统连入，不能把此处的输出一律理解为百分比。
      settings: AttributesFormatString=Range（限幅或范围）
  Relational Operator1 : RelationalOperator  Operator===  OutDataTypeStr=boolean  InputSameDT=off
      settings: AttributesFormatString=Relational Operator1（关系比较运算1）
  Relational Operator2 : RelationalOperator  OutDataTypeStr=boolean  InputSameDT=off
      settings: AttributesFormatString=Relational Operator2（关系比较运算2）
  Switch : Switch  Criteria=u2 ~= 0  SaturateOnIntegerOverflow=off  InputSameDT=off
      settings: AttributesFormatString=Switch（开关选择）
  Switch1 : Switch  Criteria=u2 ~= 0  SaturateOnIntegerOverflow=off  InputSameDT=off
      settings: AttributesFormatString=Switch（开关选择）
  Time Delay1 : UnitDelay  SampleTime=-1  HasFrameUpgradeWarning=on
      settings: AttributesFormatString=Time Delay1（时间延迟1）
  Time Delay8 : UnitDelay  SampleTime=-1  HasFrameUpgradeWarning=on
      settings: AttributesFormatString=Time Delay8（时间延迟8）
  S_Eblast_Cycle : Outport
      settings: AttributesFormatString=S_Eblast_Cycle（副油阀周期计数（每计数2毫秒））
  S_Eblast_Open : Outport  Port=2
      settings: AttributesFormatString=S_Eblast_Open（副油阀开通计数（每计数2毫秒））
  S_Eblast_Enable : Outport  Port=3
      settings: AttributesFormatString=S_Eblast_Enable（副油阀驱动使能）
  wires:
  Constant5/1 -> S_Eblast_Cycle/1
  S_COMM_Data6/1 -> Data Type Conversion2/1
  Data Type Conversion2/1 -> Product3/1
  Time Delay8/1 -> Switch/3
  Constant2/1 -> Product3/2
  Constant7/1 -> Product3/3
  S_Instr/1 -> Relational Operator1/2
  N1r_idle1/1 -> Relational Operator1/1
  Constant3/1 -> Range/2(Max)
  Constant1/1 -> Range/3(Min)
  Product3/1 -> Relational Operator2/1, Range/1(In)
  Relational Operator1/1 -> Logical Operator/1
  S_Flag_rs_suc/1 -> Logical Operator/2
  Constant8/1 -> Relational Operator2/2
  Range/1(Out) -> Data Type Conversion1/1
  Relational Operator2/1 -> Switch1/1
  Logical Operator/1 -> Switch/2, Switch1/2
  Time Delay1/1 -> Switch1/3
  Data Type Conversion1/1 -> Switch/1
  Switch1/1 -> Data Type Conversion3/1, Time Delay1/1
  Switch/1 -> Time Delay8/1, S_Eblast_Open/1
  Data Type Conversion3/1 -> S_Eblast_Enable/1

== system turbo_controller/CLM/Manual/Firework_Control ==
  note: 手动设置点火器并记住上次选择
      |
      | 先检查有效接收标志和点火器设置命令是否同时成立。成立时，Data6≥1表示开，Data6<1表示关；否
      | 则使用单拍延迟保存的旧值。输出又送回延迟块，因此一次有效命令会持续生效，直到下一次有效点火
      | 命令修改它。
      |
      | 这里输出的是点火许可，最终的9拍开、1拍关节奏由BoardOutput中的点火时序模块产生。本处不直接
      | 生成GPIO脉冲。
  S_Flag_rs_suc : Inport
      settings: AttributesFormatString=S_Flag_rs_suc（标志接收状态成功或有效）
  S_Instr : Inport  Port=2
      settings: AttributesFormatString=S_Instr（指令）
  S_COMM_Data6 : Inport  Port=3
      settings: AttributesFormatString=S_COMM_Data6（通信数据6）
  Constant8 : Constant  OutDataTypeStr=uint8
      settings: AttributesFormatString=Constant8（常量8）
  Data Type Conversion1 : DataTypeConversion  OutDataTypeStr=uint8  SaturateOnIntegerOverflow=off  RndMeth=Floor
      settings: AttributesFormatString=Data Type Conversion1（数据类型转换1）
  Logical Operator : Logic  AllPortsSameDT=off  OutDataTypeStr=boolean
      settings: AttributesFormatString=Logical Operator（逻辑运算）
  N1r_idle1 : Constant  Value=PG_Instr_FireWorkSet  OutDataTypeStr=single  SampleTime=-1
      settings: AttributesFormatString=N1r_idle1（一级转速归一化值慢车1）
  Relational Operator1 : RelationalOperator  Operator===  OutDataTypeStr=boolean  InputSameDT=off
      settings: AttributesFormatString=Relational Operator1（关系比较运算1）
  Relational Operator2 : RelationalOperator  OutDataTypeStr=boolean  InputSameDT=off
      settings: AttributesFormatString=Relational Operator2（关系比较运算2）
  Switch : Switch  Criteria=u2 ~= 0  SaturateOnIntegerOverflow=off  InputSameDT=off
      settings: AttributesFormatString=Switch（开关选择）
  Time Delay8 : UnitDelay  SampleTime=-1  HasFrameUpgradeWarning=on
      settings: AttributesFormatString=Time Delay8（时间延迟8）
  S_SWO_Firework : Outport
      settings: AttributesFormatString=S_SWO_Firework（点火器使能（1开））
  wires:
  S_Instr/1 -> Relational Operator1/2
  S_Flag_rs_suc/1 -> Logical Operator/2
  N1r_idle1/1 -> Relational Operator1/1
  Relational Operator1/1 -> Logical Operator/1
  Switch/1 -> Time Delay8/1, S_SWO_Firework/1
  Relational Operator2/1 -> Data Type Conversion1/1
  S_COMM_Data6/1 -> Relational Operator2/1
  Constant8/1 -> Relational Operator2/2
  Time Delay8/1 -> Switch/3
  Data Type Conversion1/1 -> Switch/1
  Logical Operator/1 -> Switch/2
